simulink model "InfusionPumpSoftwareModel"  (R2022b)
settings: Solver=FixedStepDiscrete  StartTime=0.0  StopTime=120  FixedStep=0.001  MaxStep=0.001  RelTol=1e-5
PreLoadFcn:
  | InitializationInsulinPump
undefined symbols (not defined in the file): reserv_str
settings Model: Creator=szhang  LastModifiedBy=ppatel
settings SolverCC: AlgebraicLoopSolver=TrustRegion
settings DataIOCC: InitialState=simState  LimitDataPoints=on  SaveFinalState=on  SaveOutput=off  SaveTime=off
settings OptimizationCC: BlockReduction=off  DefaultParameterBehavior=Inlined  UseDivisionForNetSlopeComputation=on  UseFloatMulNetSlope=on  InlineInvariantSignals=on  PassReuseOutputArgsAs=Individual arguments  EfficientFloat2IntCast=on  LifeSpan=inf  EfficientTunableParamExpr=on
settings DebuggingCC: SignalInfNanChecking=error  SignalRangeChecking=error  ReadBeforeWriteMsg=EnableAllAsError  WriteAfterWriteMsg=EnableAllAsError  WriteAfterReadMsg=EnableAllAsError  AlgebraicLoopMsg=error  ArtificialAlgebraicLoopMsg=error  SaveWithDisabledLinksMsg=error  SaveWithParameterizedLinksMsg=error  BlockPriorityViolationMsg=error  SolverPrmCheckMsg=error  InheritedTsInSrcMsg=error  SingleTaskRateTransMsg=error  TasksWithSamePriorityMsg=error  SigSpecEnsureSampleTimeMsg=error  CheckMatrixSingularityMsg=error  IntegerOverflowMsg=error  ParameterUnderflowMsg=error  ParameterPrecisionLossMsg=none  ParameterTunabilityLossMsg=error  UnderSpecifiedDataTypeMsg=error  UnnecessaryDatatypeConvMsg=warning  VectorMatrixConversionMsg=error  SignalLabelMismatchMsg=error  UnconnectedInputMsg=error  UnconnectedOutputMsg=error  UnconnectedLineMsg=error  SFcnCompatibilityMsg=error  UniqueDataStoreMsg=error  BusObjectLabelMismatch=error  RootOutportRequireBusObject=error  AssertControl=DisableAll  ModelReferenceIOMsg=error  ModelReferenceIOMismatchMessage=error  UnknownTsInhSupMsg=error  ModelReferenceDataLoggingMessage=error  StateNameClashWarn=warning  StrictBusMsg=ErrorOnBusTreatedAsVector  NonBusSignalsTreatedAsBus=error  SFInvalidInputDataAccessInChartInitDiag=error  SFTransitionOutsideNaturalParentDiag=error  SFUnreachableExecutionPathDiag=error  SFUndirectedBroadcastEventsDiag=error  SFTransitionActionBeforeConditionDiag=error  SFTemporalDelaySmallerThanSampleTimeDiag=error  SFSelfTransitionDiag=error  SFExecutionAtInitializationDiag=error  IntegerSaturationMsg=error  VariantConditionMismatch=error
settings HardwareCC: ProdLongLongMode=on
settings ModelReferenceCC: EnableRefExpFcnMdlSchedulingChecks=on  PropagateVarSize=During execution  PropagateSignalLabelsOutOfModel=off
settings SFSimCC: SimUseLocalCustomCode=off  CompileTimeRecursionLimit=0  EnableRuntimeRecursion=off  MATLABDynamicMemAlloc=off  CustomCodeUndefinedFunction=UseInterfaceOnly
settings RTWCC: Description=Embedded Coder  SystemTargetFile=ert.tlc  GenCodeOnly=on  PackageGeneratedCodeAndArtifacts=on  PackageName=packagetest  TemplateMakefile=ert_default_tmf  GenerateReport=on  RTWUseLocalCustomCode=off  IncludeHyperlinkInReport=on  LaunchReport=on  PortableWordSizes=on  GenerateTraceInfo=on  GenerateTraceReport=on  GenerateTraceReportSl=on  GenerateTraceReportSf=on  GenerateTraceReportEml=on  GenerateCodeMetricsReport=on
settings CodeAppCC: ForceParamTrailComments=on  IgnoreCustomStorageClasses=off  OperatorAnnotations=on  SimulinkDataObjDesc=on  SFDataObjDesc=on  MATLABFcnDesc=on  MangleLength=4  CustomSymbolStrGlobalVar=rt$N$M  CustomSymbolStrType=$N$M  CustomSymbolStrFcn=$N$M$F  CustomSymbolStrMacro=$N$M  InsertBlockDesc=on  StateflowObjectComments=on  MATLABSourceComments=on  ReqsInCode=on
settings ERTTargetCC: UtilityFuncGeneration=Shared location  MultiwordLength=2048  GenerateSampleERTMain=on  IncludeMdlTerminateFcn=off  CombineSignalStateStructs=on  SuppressErrorStatus=on  SupportAbsoluteTime=off  SupportNonFinite=off  SupportComplex=off  ParenthesesLevel=Maximum  CastingMode=Standards  GenerateSharedConstants=off  InlinedParameterPlacement=NonHierarchical  ERTCustomFileTemplate=example_file_process.tlc  ERTFilePackagingFormat=CompactWithDataFile  PreserveExpressionOrder=on  EnableSignedLeftShifts=off  EnableSignedRightShifts=off
settings ConfigComp: CovEnable=on  CovScope=ReferencedModels  CovIncludeTopModel=off  CovMetricSettings=dcmw  CovHTMLOptions=-sRT=1 -sVT=0 -aTS=1 -bRG=1 -bTC=1 -hTR=0 -nFC=0 -nFD=1 -scm=1 -bcm=1 -xEv=0 -xEM=0  CovSaveCumulativeToWorkspaceVar=on  CovSaveSingleToWorkspaceVar=on  CovCumulativeReport=on  CovModelRefEnable=on  CovExternalEMLEnable=off  CovSFcnEnable=off  DVTestSuiteOptimization=CombinedObjectives (Nonlinear Extended)  DVDesignMinMaxCheck=on  DVHarnessSource=Signal Editor  PSOpenProjectManager=on  PSResultDir=ps_results_$ModelName$  PSAutoStubLUT=on
settings SimscapeCC: SimscapeNormalizeSystem=off  SimscapeLogType=all  SimscapeLogLimitData=off

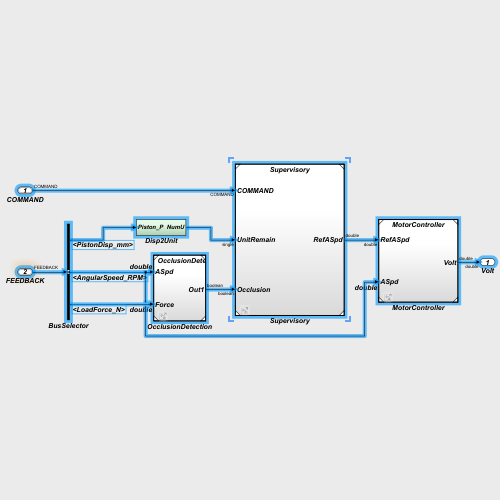
[thumbnail: Simulink's stored preview of the top-level diagram]
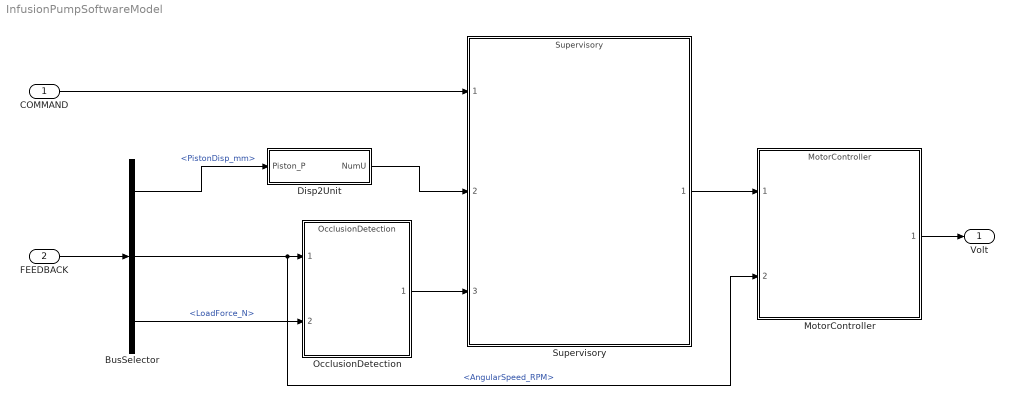
== system InfusionPumpSoftwareModel ==
  COMMAND : Inport  OutDataTypeStr=Bus: COMMAND  PortDimensions=1  SampleTime=0.001  BusOutputAsStruct=on
  FEEDBACK : Inport  Port=2  OutDataTypeStr=Bus: FEEDBACK  PortDimensions=1  SampleTime=0.001  BusOutputAsStruct=on
  BusSelector : BusSelector  OutputSignals=PistonDisp_mm,AngularSpeed_RPM,LoadForce_N
  Disp2Unit : Subsystem
  MotorController : ModelReference  ModelNameDialog=MotorController  SimulationMode=Normal  ModelReferenceVersion=11.6
  OcclusionDetection : ModelReference  ModelNameDialog=OcclusionDetection.slx  SimulationMode=Normal  ModelReferenceVersion=9.8
  Supervisory : ModelReference  ModelNameDialog=Supervisory  SimulationMode=Normal  ModelReferenceVersion=11.11
  Volt : Outport  OutMin=-20  OutMax=20  OutDataTypeStr=double  PortDimensions=1  SampleTime=[0.001,0]  VectorParamsAs1DForOutWhenUnconnected=off
  wires:
  Disp2Unit/1(NumU) -> Supervisory/2
  Supervisory/1 -> MotorController/1
  BusSelector/2 -> MotorController/2, OcclusionDetection/1  "<AngularSpeed_RPM>"
  MotorController/1 -> Volt/1
  BusSelector/3 -> OcclusionDetection/2  "<LoadForce_N>"
  FEEDBACK/1 -> BusSelector/1
  BusSelector/1 -> Disp2Unit/1(Piston_P)  "<PistonDisp_mm>"
  OcclusionDetection/1 -> Supervisory/3
  COMMAND/1 -> Supervisory/1

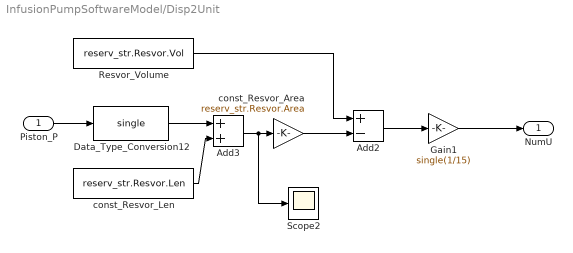
== system InfusionPumpSoftwareModel/Disp2Unit ==
  Piston_P : Inport  OutMin=-30  OutMax=0
  Add2 : Sum  Inputs=+-
  Add3 : Sum
  Data_Type_Conversion12 : DataTypeConversion  OutDataTypeStr=single  SaturateOnIntegerOverflow=off  RndMeth=Floor
  Gain1 : Gain  Gain=single(1/15)
  Resvor_Volume : Constant  Value=reserv_str.Resvor.Vol  OutDataTypeStr=single
  Scope2 : Scope
  const_Resvor_Area : Gain  Gain=reserv_str.Resvor.Area  ParamDataTypeStr=single
  const_Resvor_Len : Constant  Value=reserv_str.Resvor.Len  OutDataTypeStr=single
  NumU : Outport  OutMin=0  OutMax=201  VectorParamsAs1DForOutWhenUnconnected=off
  wires:
  Resvor_Volume/1 -> Add2/1
  const_Resvor_Len/1 -> Add3/2
  const_Resvor_Area/1 -> Add2/2
  Add2/1 -> Gain1/1
  Gain1/1 -> NumU/1
  Add3/1 -> const_Resvor_Area/1, Scope2/1
  Piston_P/1 -> Data_Type_Conversion12/1
  Data_Type_Conversion12/1 -> Add3/1
